simulink model "finalmodel1"  (R2024b)
(part 7 of 9)

Yingli Energy (China) YL345D-36b | Yingli Energy (China) YL350D-36b | Yingli Energy (China) YL355D-36b | Yingli Energy (China) YL360D-36b | YOCASOL PCA200-C04 | YOCASOL PCB200-C21 | YOCASOL PCA205-C04 | YOCASOL PCB205-C21 | YOCASOL PCA210-C04 | YOCASOL PCB210-C21 | Yunnan Tianda Photovoltaic TD160M5 | Yunnan Tianda Photovoltaic TD165M5 | Yunnan Tianda Photovoltaic TD170M5 | Yunnan Tianda Photovoltaic TD175M5 | Yunnan Tianda Photovoltaic TD180M5 | Zebra Energy ZBR-185M5 | Zebra Energy ZBR-190M5 | Zebra Energy ZBR-195M5 | Zebra Energy ZBR-200M5 | Zebra Energy ZBR-200P | Zebra Energy ZBR-210P | Zebra Energy ZBR-220P | Zebra Energy ZBR-230P | Zebra Energy ZBR-235P | Zebra Energy ZBR-240MA | Zebra Energy ZBR-240PA | Zebra Energy ZBR-245MA | Zebra Energy ZBR-250MA | Zebra Energy ZBR-250P | Zebra Energy ZBR-255M | Zebra Energy ZBR-260P | Zebra Energy ZBR-270P | Zebra Energy ZBR-280P | Zebra Energy ZBR-285P | Zebra Energy ZBR-290M | Zebra Energy ZBR-290P | Zebra Energy ZBR-295M | Zebra Energy ZBR-295P | Zebra Energy ZBR-300M | Zebra Energy ZBR-300P | Zebra Energy ZBR-305M | Zebra Energy ZBR-310M | Zerquest Solar Zp170 | Zhangjiagang City SEG PV SEGM5-72 170W | Zhangjiagang City SEG PV SEGM5-72 175W | Zhangjiagang City SEG PV SEGM5-72 180W | Zhangjiagang City SEG PV SEGM5-72 185W | Zhangjiagang City SEG PV SEGM5-72 190W | Zhangjiagang City SEG PV SEGM6-54 190W | Zhangjiagang City SEG PV SEGM5-72 195W | Zhangjiagang City SEG PV SEGM6-54 195W | Zhangjiagang City SEG PV SEGM6-54 200W | Zhangjiagang City SEG PV SEGM6-60 200W | Zhangjiagang City SEG PV SEGM6-54 205W | Zhangjiagang City SEG PV SEGM6-60 205W | Zhangjiagang City SEG PV SEGM6-54 210W | Zhangjiagang City SEG PV SEGM6-60 210W | Zhangjiagang City SEG PV SEGM6-60 215W | Zhangjiagang City SEG PV SEGM6-60 220W | Zhangjiagang City SEG PV SEGM6-60 225W | Zhangjiagang City SEG PV SEGM5-96 230W | Zhangjiagang City SEG PV SEGM6-60 230W | Zhangjiagang City SEG PV SEGM5-96 235W | Zhangjiagang City SEG PV SEGM6-60 235W | Zhangjiagang City SEG PV SEGM5-96 240W | Zhangjiagang City SEG PV SEGM6-60 240W | Zhangjiagang City SEG PV SEGM5-96 245W | Zhangjiagang City SEG PV SEGM5-96 250W | Zhangjiagang City SEG PV SEGM5-96 255W | Zhangjiagang City SEG PV SEGM6-72 255W | Zhangjiagang City SEG PV SEGP6-72 255W | Zhangjiagang City SEG PV SEGM6-72 260W | Zhangjiagang City SEG PV SEGP6-72 260W | Zhangjiagang City SEG PV SEGM6-72 265W | Zhangjiagang City SEG PV SEGP6-72 265W | Zhangjiagang City SEG PV SEGM6-72 270W | Zhangjiagang City SEG PV SEGP6-72 270W | Zhangjiagang City SEG PV SEGM6-72 275W | Zhangjiagang City SEG PV SEGP6-72 275W | Zhangjiagang City SEG PV SEGM6-72 280W | Zhangjiagang City SEG PV SEGP6-72 280W | Zhangjiagang City SEG PV SEGM6-72 285W | Zhangjiagang City SEG PV SEGP6-72 285W | Zhangjiagang City SEG PV SEGM6-72 290W | Zhangjiagang City SEG PV SEGP6-72 290W | Zhangjiagang City SEG PV SEGM6-72 295W | Zhangjiagang City SEG PV SEGP6-72 295W | Zhangjiagang City SEG PV SEGM6-72 300W | Zhangjiagang City SEG PV SEGP6-72 300W | Zhangjiagang City Sunlink PV SEGP6-54-195 | Zhangjiagang City Sunlink PV SEGP6-54-200 | Zhangjiagang City Sunlink PV SEGP6-54-205 | Zhangjiagang City Sunlink PV SEGP6-60-220 | Zhangjiagang City Sunlink PV SEGP6-60-225 | Zhangjiagang City Sunlink PV SEGP6-60-230 | Zhejiang ERA Solar Technology ESPSA-170 | Zhejiang ERA Solar Technology ESPSA-175 | Zhejiang ERA Solar Technology ESPSA-180 | Zhejiang Global Photovoltaic Technology GSM-155 | Zhejiang Global Photovoltaic Technology GSM-160 | Zhejiang Global Photovoltaic Technology GSM-165 | Zhejiang Global Photovoltaic Technology GSM-170 | Zhejiang Global Photovoltaic Technology GSM-175 | Zhejiang Global Photovoltaic Technology GSM-180 | Zhejiang Global Photovoltaic Technology GSP-230 | Zhejiang Global Photovoltaic Technology GSM-235 | Zhejiang Global Photovoltaic Technology GSP-235 | Zhejiang Global Photovoltaic Technology GSM-240 | Zhejiang Global Photovoltaic Technology GSP-240 | Zhejiang Global Photovoltaic Technology GSM-245 | Zhejiang Global Photovoltaic Technology GSM-250 | Zhejiang Global Photovoltaic Technology GSP-265 | Zhejiang Global Photovoltaic Technology GSP-270 | Zhejiang Global Photovoltaic Technology GSM-275 | Zhejiang Global Photovoltaic Technology GSP-275 | Zhejiang Global Photovoltaic Technology GSM-280 | Zhejiang Global Photovoltaic Technology GSP-280 | Zhejiang Global Photovoltaic Technology GSM-285 | Zhejiang Global Photovoltaic Technology GSP-285 | Zhejiang Global Photovoltaic Technology GSM-290 | Zhejiang Global Photovoltaic Technology GSM-295 | Zhejiang Global Photovoltaic Technology GSM-300 | Zhejiang Global Photovoltaic Technology GSM-305 | Zhejiang Guangyi Optical Energy Technology GYP-150M | Zhejiang Guangyi Optical Energy Technology GYP-170P | Zhejiang Guangyi Optical Energy Technology GYP-175P | Zhejiang Guangyi Optical Energy Technology GYP-180M | Zhejiang Guangyi Optical Energy Technology GYP-180P | Zhejiang Guangyi Optical Energy Technology GYP-185M | Zhejiang Guangyi Optical Energy Technology GYP-185P | Zhejiang Guangyi Optical Energy Technology GYP-190P | Zhejiang Guangyi Optical Energy Technology GYP-200P | Zhejiang Guangyi Optical Energy Technology GYP-210P | Zhejiang Guangyi Optical Energy Technology GYP-220P | Zhejiang Guangyi Optical Energy Technology GYP-225P | Zhejiang Guangyi Optical Energy Technology GYP-230M | Zhejiang Guangyi Optical Energy Technology GYP-230P | Zhejiang Guangyi Optical Energy Technology GYP-235M | Zhejiang Guangyi Optical Energy Technology GYP-240M | Zhejiang Guangyi Optical Energy Technology GYP-245M | Zhejiang Guangyi Optical Energy Technology GYP-250M | Zhejiang Guangyi Optical Energy Technology GYP-265P | Zhejiang Guangyi Optical Energy Technology GYP-270M | Zhejiang Guangyi Optical Energy Technology GYP-270P | Zhejiang Guangyi Optical Energy Technology GYP-280M | Zhejiang Guangyi Optical Energy Technology GYP-280P | Zhejiang Guangyi Optical Energy Technology GYP-285P | Zhejiang Guangyi Optical Energy Technology GYP-290M | Zhejiang Jingshang New Energy Technology STS-6M-145P-36 | Zhejiang Jingshang New Energy Technology STS-6M-150P-36 | Zhejiang Jingshang New Energy Technology STS-6M-155P-36 | Zhejiang Jingshang New Energy Technology STS-6M-185P-48 | Zhejiang Jingshang New Energy Technology STS-6M-190P-48 | Zhejiang Jingshang New Energy Technology STS-6M-195P-48 | Zhejiang Jingshang New Energy Technology STS-6M-200P-48 | Zhejiang Jingshang New Energy Technology STS-6M-210P-54 | Zhejiang Jingshang New Energy Technology STS-6M-215P-54 | Zhejiang Jingshang New Energy Technology STS-6M-220P-54 | Zhejiang Jingshang New Energy Technology STS-6M-225P-54 | Zhejiang Jingshang New Energy Technology STS-6M-230P-54 | Zhejiang Jingshang New Energy Technology STS-6M-235P-60 | Zhejiang Jingshang New Energy Technology STS-6M-240P-60 | Zhejiang Jingshang New Energy Technology STS-6M-245P-60 | Zhejiang Jingshang New Energy Technology STS-6M-250P-60 | Zhejiang Jingshang New Energy Technology STS-6M-255P-60 | Zhejiang Jingshang New Energy Technology STS-6M-260P-60 | Zhejiang Jingshang New Energy Technology STS-6M-265P-60 | Zhejiang Jingshang New Energy Technology STS-6M-270P-72 | Zhejiang Jingshang New Energy Technology STS-6M-275P-72 | Zhejiang Jingshang New Energy Technology STS-6M-280P-72 | Zhejiang Jingshang New Energy Technology STS-6M-285P-72 | Zhejiang Jingshang New Energy Technology STS-6M-290P-72 | Zhejiang Jingshang New Energy Technology STS-6M-295P-72 | Zhejiang Jingshang New Energy Technology STS-6M-300P-72 | Zhejiang Jingshang New Energy Technology STS-6M-305P-72 | Zhejiang Jingshang New Energy Technology STS-6M-310P-72 | Zhejiang Jingshang New Energy Technology STS-6M-315P-72 | Zhejiang Jingshang New Energy Technology STS-6M-320P-72 | Zhejiang Jiutai New Energy JTM175-72M | Zhejiang Jiutai New Energy JTM180-72M | Zhejiang Jiutai New Energy JTM185-72M | Zhejiang Jiutai New Energy JTM200-60P | Zhejiang Jiutai New Energy JTM205-60P | Zhejiang Jiutai New Energy JTM210-60P | Zhejiang Jiutai New Energy JTM215-60P | Zhejiang Jiutai New Energy JTM220-60P | Zhejiang Jiutai New Energy JTM225-60P | Zhejiang Jiutai New Energy JTM230-60P | Zhejiang Jiutai New Energy JTM235-60P | Zhejiang Jiutai New Energy JTM240-60P | Zhejiang Jiutai New Energy JTM270-72P | Zhejiang Jiutai New Energy JTM275-72P | Zhejiang Jiutai New Energy JTM280-72P | Zhejiang Jiutai New Energy JTM285-72P | Zhejiang Kingdom Solar Energy Technic KD-M160 | Zhejiang Kingdom Solar Energy Technic KD-M165 | Zhejiang Kingdom Solar Energy Technic KD-M170 | Zhejiang Kingdom Solar Energy Technic KD-M175 | Zhejiang Kingdom Solar Energy Technic KD-M180 | Zhejiang Kingdom Solar Energy Technic KD-M185 | Zhejiang Kingdom Solar Energy Technic KD-M190 | Zhejiang Kingdom Solar Energy Technic KD-M195 | Zhejiang Kingdom Solar Energy Technic KD-M200 | Zhejiang Kingdom Solar Energy Technic KD-P200 | Zhejiang Kingdom Solar Energy Technic KD-P205 | Zhejiang Kingdom Solar Energy Technic KD-P210 | Zhejiang Kingdom Solar Energy Technic KD-P215 | Zhejiang Kingdom Solar Energy Technic KD-P220 | Zhejiang Kingdom Solar Energy Technic KD-P225 | Zhejiang Kingdom Solar Energy Technic KD-P230 | Zhejiang Kingdom Solar Energy Technic KD-P235 | Zhejiang Kingdom Solar Energy Technic KD-P240 | Zhejiang Kingdom Solar Energy Technic KD-P245 | Zhejiang Kingdom Solar Energy Technic KD-P250 | Zhejiang Kingdom Solar Energy Technic KD-P255 | Zhejiang Kingdom Solar Energy Technic KD-P260 | Zhejiang Kingdom Solar Energy Technic KD-P265 | Zhejiang Kingdom Solar Energy Technic KD-P270 | Zhejiang Kingdom Solar Energy Technic KD-P275 | Zhejiang Kingdom Solar Energy Technic KD-P280 | Zhejiang Kingdom Solar Energy Technic KD-P285 | Zhejiang Kingdom Solar Energy Technic KD-P290 | Zhejiang Kingdom Solar Energy Technic KD-P295 | Zhejiang Kingdom Solar Energy Technic KD-P300 | Zhejiang Shinew Photoelectronic Technology XH-72M-185 | Zhejiang Shinew Photoelectronic Technology XH-72M-190 | Zhejiang Shinew Photoelectronic Technology XH-60P-230 | Zhejiang Shinew Photoelectronic Technology XH-60P-235 | Zhejiang Shinew Photoelectronic Technology XH-72P-280 | ZheJiang SOCO Technology SC180M-24/P | ZheJiang SOCO Technology SC230M-24/J | ZheJiang SOCO Technology SC230P-24/B | ZheJiang SOCO Technology SC275P-24/A | ZheJiang SOCO Technology SC280M-24/H | Zhejiang Sunflower Light Energy Science & Technology SF125x125-72-M-150W | Zhejiang Sunflower Light Energy Science & Technology SF125x125-72-M-155W | Zhejiang Sunflower Light Energy Science & Technology SF125x125-72-M-160W | Zhejiang Sunflower Light Energy Science & Technology SF125x125-72-M-165W | Zhejiang Sunflower Light Energy Science & Technology SF125x125-72-M-170W | Zhejiang Sunflower Light Energy Science & Technology SF125x125-72-M-175W | Zhejiang Sunflower Light Energy Science & Technology SF125x125-72-M-180W | Zhejiang Sunflower Light Energy Science & Technology SF125x125-72-M-185W | Zhejiang Sunflower Light Energy Science & Technology SF156x156-60-M-200W | Zhejiang Sunflower Light Energy Science & Technology SF156x156-60-P-200W | Zhejiang Sunflower Light Energy Science & Technology SF156x156-60-M-205W | Zhejiang Sunflower Light Energy Science & Technology SF156x156-60-P-205W | Zhejiang Sunflower Light Energy Science & Technology SF156x156-60-M-210W | Zhejiang Sunflower Light Energy Science & Technology SF156x156-60-P-210W | Zhejiang Sunflower Light Energy Science & Technology SF156x156-60-M-215W | Zhejiang Sunflower Light Energy Science & Technology SF156x156-60-P-215W | Zhejiang Sunflower Light Energy Science & Technology SF156x156-60-M-220W | Zhejiang Sunflower Light Energy Science & Technology SF156x156-60-P-220W | Zhejiang Sunflower Light Energy Science & Technology SF156x156-60-M-225W | Zhejiang Sunflower Light Energy Science & Technology SF156x156-60-P-225W | Zhejiang Sunflower Light Energy Science & Technology SF156x156-60-M-230W | Zhejiang Sunflower Light Energy Science & Technology SF156x156-60-P-230W | Zhejiang Sunflower Light Energy Science & Technology SF156x156-60-M-235W | Zhejiang Sunflower Light Energy Science & Technology SF156x156-60-M-240W | Zhejiang Trunsun Solar Co._ Ltd. TSP255-60 | Zhejiang Trunsun Solar Co._ Ltd. TSM260-60 | Zhejiang Trunsun Solar Co._ Ltd. TSP260-60 | Zhejiang Trunsun Solar Co._ Ltd. TSM265-60 | Zhejiang Trunsun Solar Co._ Ltd. TSP265-60 | Zhejiang Trunsun Solar Co._ Ltd. TSM270-60 | Zhejiang Trunsun Solar Co._ Ltd. TSP270-60 | Zhejiang Trunsun Solar Co._ Ltd. TSM275-60 | Zhejiang Trunsun Solar Co._ Ltd. TSP275-60 | Zhejiang Trunsun Solar Co._ Ltd. TSP305-72 | Zhejiang Trunsun Solar Co._ Ltd. TSM310-72 | Zhejiang Trunsun Solar Co._ Ltd. TSP310-72 | Zhejiang Trunsun Solar Co._ Ltd. TSM315-72 | Zhejiang Trunsun Solar Co._ Ltd. TSP315-72 | Zhejiang Trunsun Solar Co._ Ltd. TSM320-72 | Zhejiang Trunsun Solar Co._ Ltd. TSP320-72 | Zhejiang Trunsun Solar Co._ Ltd. TSM325-72 | Zhejiang Trunsun Solar Co._ Ltd. TSP325-72 | Zhejiang Trunsun Solar Co._ Ltd. TSM330-72 | Zhejiang Trunsun Solar Co._ Ltd. TSP330-72 | Zhejiang Trunsun Solar Co._ Ltd. TSP335-72 | Zhejiang Wanxiang Solar WXS175P | Zhejiang Wanxiang Solar WXS175S | Zhejiang Wanxiang Solar WXS180P | Zhejiang Wanxiang Solar WXS180S | Zhejiang Wanxiang Solar WXS185P | Zhejiang Wanxiang Solar WXS185S | Zhejiang Wanxiang Solar WXS190P | Zhejiang Wanxiang Solar WXS200P | Zhejiang Wanxiang Solar WXS205P | Zhejiang Wanxiang Solar WXS210P | Zhejiang Wanxiang Solar WXS215P | Zhejiang Wanxiang Solar WXS220P | Zhejiang Wanxiang Solar WXS225P | Zhejiang Wanxiang Solar WXS230P | Zhejiang Wanxiang Solar WXS235P | Zhejiang Wanxiang Solar WXS240P | Zhejiang Wanxiang Solar WXS245P | Zhejiang Wanxiang Solar WXS250P | Zhejiang Wanxiang Solar WXS255P | Zhejiang Wanxiang Solar WXS260P | Zhejiang Wanxiang Solar WXS265P | Zhejiang Wanxiang Solar WXS270P | Zhejiang Wanxiang Solar WXS275P | Zhejiang Wanxiang Solar WXS280P | Znshine PV-Tech ZXM5-72-175/MS | Znshine PV-Tech ZXM5-72-180/MS | Znshine PV-Tech ZXM5-72-185/MS | Znshine PV-Tech ZXM5-72-190/MS | Znshine PV-Tech ZXM5-72-195/MS | Znshine PV-Tech ZXM5-72-200/MS | Znshine PV-Tech ZXP6-60-220/P | Znshine PV-Tech ZXP6-60-225/P | Znshine PV-Tech ZXP6-60-230/P | Znshine PV-Tech ZXP6-60-235/P | Znshine PV-Tech ZXP6-D60-235/P | Znshine PV-Tech ZXM6-D60-240/M | Znshine PV-Tech ZXP6-60-240/P | Znshine PV-Tech ZXP6-D60-240/P | Znshine PV-Tech ZXM5-96-245/MS | Znshine PV-Tech ZXM6-D60-245/M | Znshine PV-Tech ZXP6-60-245/P | Znshine PV-Tech ZXP6-D60-245/P | Znshine PV-Tech ZXM5-96-250/MS | Znshine PV-Tech ZXM6-D60-250/M | Znshine PV-Tech ZXP6-D60-250/P | Znshine PV-Tech ZXM5-96-255/MS | Znshine PV-Tech ZXM6-D60-255/M | Znshine PV-Tech ZXP6-D60-255/P | Znshine PV-Tech ZXM5-96-260/MS | Znshine PV-Tech ZXM6-D60-260/M | Znshine PV-Tech ZXM5-96-265/MS | Znshine PV-Tech ZXP6-72-265/P | Znshine PV-Tech ZXM5-96-270/MS | Znshine PV-Tech ZXP6-72-270/P | Znshine PV-Tech ZXM5-96-275/MS | Znshine PV-Tech ZXP6-72-275/P | Znshine PV-Tech ZXP6-72-280/P | Znshine PV-Tech ZXP6-72-285/P | Znshine PV-Tech ZXP6-72-290/P | Znshine PV-Tech ZXP6-72-295/P | Zytech Engineering Technology ZT170S | Zytech Engineering Technology ZT175S | Zytech Engineering Technology ZT180S | Zytech Engineering Technology ZT185S | Zytech Engineering Technology ZT190S | Zytech Solar ZT145P | Zytech Solar ZT150P | Zytech Solar ZT155P | Zytech Solar ZT185P | Zytech Solar ZT190P | Zytech Solar ZT195P | Zytech Solar ZT200P | Zytech Solar ZT210P | Zytech Solar ZT215P | Zytech Solar ZT220P | Zytech Solar ZT225P | Zytech Solar ZT230P | Zytech Solar ZT235P | Zytech Solar ZT240P | Zytech Solar ZT245P | Zytech Solar ZT250P | Zytech Solar ZT255P | Zytech Solar ZT260P | Zytech Solar ZT265P | Zytech Solar ZT270P | Zytech Solar ZT275P | Zytech Solar ZT280P | Zytech Solar ZT285P | Zytech Solar ZT290P | Zytech Solar ZT295P | Zytech Solar ZT300P | Zytech Solar ZT305P | Zytech Solar ZT310P | Zytech Solar ZT315P | Zytech Solar ZT320P
      mask Callback ModuleName: PVArrayCback(gcb)
      mask Callback RobustModel: PVArrayCback(gcb)
      mask Callback BAL: PVArrayCback(gcb)
      mask DialogControl ParameterTabVar0 Prompt: Parameters
      mask DialogControl ArrayData Prompt: Array data
      mask DialogControl Display Prompt: Display  I-V and P-V characteristics of ...
      mask DialogControl PlotButton Prompt: Plot
      mask DialogControl PlotButton Callback: PVArrayPlot(gcb,'detailed')
      mask DialogControl ManufacturerData Prompt: Module data
      mask DialogControl ModelParameters Prompt: Model parameters
      mask DialogControl Advanced Prompt: Advanced
      mask Display:
      | port_label('input',1,'Ir')
      | switch WantBlockChoice{1}
      |     case 'Discrete DSS Diode Rsh'
      |     otherwise
      |         port_label('input',2,'T')
      | end
      | 
      | port_label('output',1,'m')
      | port_label('output',1,'m')
      | port_label('Rconn',1,'+')
      | port_label('Rconn',2,'-')
  PWM Generator (2-Level) : spsPWMGenerator2LevelLib/PWM Generator (2-Level)  ModulatorType=Three-phase bridge (6 pulses)  ModulatorMode=Synchronized  Fc=27*60  Pc=90  nF=27  MinMax="[ -1  1 ]"  SamplingTechnique=Natural  ModulatingSignals=off  m=0.8  Freq=60  Phase=0  Ts=SampleTime  ShowCarrierOutport=off
      link override Modulator type/One Three Phase Bridge/P: SampleTime=SampleTime
      link override P: SampleTime=SampleTime
      link override Reference signal/External/Uref: SampleTime=SampleTime
      link override Uref: SampleTime=SampleTime
      link override wt: SampleTime=SampleTime
  "PWM Generator (DC - DC) " : spsPWMGeneratorDCDCLib/PWM Generator (DC-DC)  Fsw=5e3  Ts=SampleTime
      link override D: SampleTime=SampleTime
      link override Sawtooth Generator: Ts=SampleTime
      link override Sawtooth Generator/Model/Constant2: SampleTime=SampleTime
      link override Sawtooth Generator/Model/Constant3: SampleTime=SampleTime
      link override Sawtooth Generator/Model/Digital Clock: SampleTime=SampleTime
  "Power (3ph, Instantaneous)" : spsPower3phInstantaneousLib/Power (3ph, Instantaneous)
  Product : Product  SampleTime=SampleTime
  Repeating Sequence1 : simulink/Sources/Repeating Sequence  rep_seq_t=[0 0.00005 0.0001]  rep_seq_y=[-1 1 -1]
  Scope : Scope
  Scope1 : Scope  NumInputPorts=2
  Scope2 : Scope  NumInputPorts=2
  Scope4 : Scope
  Scope5 : Scope  NumInputPorts=2
  Signal Builder2 : Subsystem  Tag=STV Subsys  Commented=on  LoadFcn=sigbuilder_block('load');  StartFcn=sigbuilder_block('start');  StopFcn=sigbuilder_block('stop');  ClipboardFcn=sigbuilder_block('clipboard');  mask(Sigbuilder block){tuvar=[0:10]}
      mask help: Simulink:masks:SigbuilderBlock_MD
      mask init:
      | if ~strcmp(get_param(bdroot(gcbh),'SimulationStatus'),'stopped') tuvar = sigbuilder_block('maskInit'); end
      settings: CopyFcn=sigbuilder_block('copy');  DeleteFcn=sigbuilder_block('delete');  ModelCloseFcn=sigbuilder_block('modelClose');  PreSaveFcn=sigbuilder_block('preSave');  PauseFcn=sigbuilder_block('pause');  ContinueFcn=sigbuilder_block('continue');  NameChangeFcn=sigbuilder_block('namechange');  OpenFcn=sigbuilder_block('open',[220.2 153.6 550.8 361.2 ]);  CloseFcn=sigbuilder_block('close');
      mask Display: plot(0, 0, 100, 100,[2, 2, 32, 32, 2], [68, 8, 8, 68, 68],[32, 2], [38, 38], [32, 19, 2],[53, 60, 44], [32, 17, 17, 2],[16, 16, 31, 31]);txt = getActiveGroup(gcbh);text(2, 100, txt,'verticalAlignment', 'top');
  Stop simulation if loss of synchronism : Stop  Commented=on
  Sum{1..3,7} (4 alike) : Sum  Inputs=|+-  SampleTime=SampleTime
  Sum{4..6,8} (4 alike) : Sum  Inputs=|++  SampleTime=SampleTime
  THD : spsTHDLib/THD  Freq=50  Ts=SampleTime
      link override In: SampleTime=SampleTime
      link override Mean: Ts=SampleTime
      link override Mean/In: SampleTime=SampleTime
      link override Mean/Mean: SampleTime=SampleTime
      link override Mean/Model/Digital  Clock: SampleTime=SampleTime
      link override Mean/Model/Discrete Variable Time Delay: Ts=SampleTime
      link override Mean/Model/Discrete Variable Time Delay/D: SampleTime=SampleTime
      link override Mean/Model/Discrete Variable Time Delay/In: SampleTime=SampleTime
      link override Mean/Model/Discrete Variable Time Delay/Out: SampleTime=SampleTime
      link override Mean/Model/Integ4: SampleTime=SampleTime
      link override Mean/Model/K1: SampleTime=SampleTime
      link override Mean/Model/K2: SampleTime=SampleTime
      link override Mean/Model/Relational Operator: SampleTime=SampleTime
      link override Mean/Model/Unit Delay: SampleTime=SampleTime
      link override Mean/Model/Unit Delay1: SampleTime=SampleTime
      link override RMS1: Ts=SampleTime
      link override RMS1/In: SampleTime=SampleTime
      link override RMS1/RMS: SampleTime=SampleTime
      link override RMS1/RMS /Fourier1: Ts=SampleTime
      link override RMS1/RMS /Fourier1/In: SampleTime=SampleTime
      link override RMS1/RMS /Fourier1/Mag: SampleTime=SampleTime
      link override RMS1/RMS /Fourier1/Mean: Ts=SampleTime
      link override RMS1/RMS /Fourier1/Mean value1: Ts=SampleTime
      link override RMS1/RMS /Fourier1/Mean value1/In: SampleTime=SampleTime
      link override RMS1/RMS /Fourier1/Mean value1/Mean: SampleTime=SampleTime
      link override RMS1/RMS /Fourier1/Mean value1/Model/Digital  Clock: SampleTime=SampleTime
      link override RMS1/RMS /Fourier1/Mean value1/Model/Discrete Variable Time Delay: Ts=SampleTime
      link override RMS1/RMS /Fourier1/Mean value1/Model/Discrete Variable Time Delay/D: SampleTime=SampleTime
      link override RMS1/RMS /Fourier1/Mean value1/Model/Discrete Variable Time Delay/In: SampleTime=SampleTime
      link override RMS1/RMS /Fourier1/Mean value1/Model/Discrete Variable Time Delay/Out: SampleTime=SampleTime
      link override RMS1/RMS /Fourier1/Mean value1/Model/Integ4: SampleTime=SampleTime
      link override RMS1/RMS /Fourier1/Mean value1/Model/K1: SampleTime=SampleTime
      link override RMS1/RMS /Fourier1/Mean value1/Model/K2: SampleTime=SampleTime
      link override RMS1/RMS /Fourier1/Mean value1/Model/Relational Operator: SampleTime=SampleTime
      link override RMS1/RMS /Fourier1/Mean value1/Model/Unit Delay: SampleTime=SampleTime
      link override RMS1/RMS /Fourier1/Mean value1/Model/Unit Delay1: SampleTime=SampleTime
      link override RMS1/RMS /Fourier1/Mean/In: SampleTime=SampleTime
      link override RMS1/RMS /Fourier1/Mean/Mean: SampleTime=SampleTime
      link override RMS1/RMS /Fourier1/Mean/Model/Digital  Clock: SampleTime=SampleTime
      link override RMS1/RMS /Fourier1/Mean/Model/Discrete Variable Time Delay: Ts=SampleTime
      link override RMS1/RMS /Fourier1/Mean/Model/Discrete Variable Time Delay/D: SampleTime=SampleTime
      link override RMS1/RMS /Fourier1/Mean/Model/Discrete Variable Time Delay/In: SampleTime=SampleTime
      link override RMS1/RMS /Fourier1/Mean/Model/Discrete Variable Time Delay/Out: SampleTime=SampleTime
      link override RMS1/RMS /Fourier1/Mean/Model/Integ4: SampleTime=SampleTime
      link override RMS1/RMS /Fourier1/Mean/Model/K1: SampleTime=SampleTime
      link override RMS1/RMS /Fourier1/Mean/Model/K2: SampleTime=SampleTime
      link override RMS1/RMS /Fourier1/Mean/Model/Relational Operator: SampleTime=SampleTime
      link override RMS1/RMS /Fourier1/Mean/Model/Unit Delay: SampleTime=SampleTime
      link override RMS1/RMS /Fourier1/Mean/Model/Unit Delay1: SampleTime=SampleTime
      link override RMS1/RMS /Fourier1/Phase: SampleTime=SampleTime
      link override RMS1/RMS /Fourier1/cos(wt): SampleTime=SampleTime
      link override RMS1/RMS /Fourier1/sin(wt): SampleTime=SampleTime
      link override RMS1/TrueRMS /Mean value: Ts=SampleTime
      link override RMS1/TrueRMS /Mean value/In: SampleTime=SampleTime
      link override RMS1/TrueRMS /Mean value/Mean: SampleTime=SampleTime
      link override RMS1/TrueRMS /Mean value/Model/Digital  Clock: SampleTime=SampleTime
      link override RMS1/TrueRMS /Mean value/Model/Discrete Variable Time Delay: Ts=SampleTime
      link override RMS1/TrueRMS /Mean value/Model/Discrete Variable Time Delay/D: SampleTime=SampleTime
      link override RMS1/TrueRMS /Mean value/Model/Discrete Variable Time Delay/In: SampleTime=SampleTime
      link override RMS1/TrueRMS /Mean value/Model/Discrete Variable Time Delay/Out: SampleTime=SampleTime
      link override RMS1/TrueRMS /Mean value/Model/Integ4: SampleTime=SampleTime
      link override RMS1/TrueRMS /Mean value/Model/K1: SampleTime=SampleTime
      link override RMS1/TrueRMS /Mean value/Model/K2: SampleTime=SampleTime
      link override RMS1/TrueRMS /Mean value/Model/Relational Operator: SampleTime=SampleTime
      link override RMS1/TrueRMS /Mean value/Model/Unit Delay: SampleTime=SampleTime
      link override RMS1/TrueRMS /Mean value/Model/Unit Delay1: SampleTime=SampleTime
      link override RMS2: Ts=SampleTime
      link override RMS2/In: SampleTime=SampleTime
      link override RMS2/RMS: SampleTime=SampleTime
      link override RMS2/RMS /Fourier1: Ts=SampleTime
      link override RMS2/RMS /Fourier1/In: SampleTime=SampleTime
      link override RMS2/RMS /Fourier1/Mag: SampleTime=SampleTime
      link override RMS2/RMS /Fourier1/Mean: Ts=SampleTime
      link override RMS2/RMS /Fourier1/Mean value1: Ts=SampleTime
      link override RMS2/RMS /Fourier1/Mean value1/In: SampleTime=SampleTime
      link override RMS2/RMS /Fourier1/Mean value1/Mean: SampleTime=SampleTime
      link override RMS2/RMS /Fourier1/Mean value1/Model/Digital  Clock: SampleTime=SampleTime
      link override RMS2/RMS /Fourier1/Mean value1/Model/Discrete Variable Time Delay: Ts=SampleTime
      link override RMS2/RMS /Fourier1/Mean value1/Model/Discrete Variable Time Delay/D: SampleTime=SampleTime
      link override RMS2/RMS /Fourier1/Mean value1/Model/Discrete Variable Time Delay/In: SampleTime=SampleTime
      link override RMS2/RMS /Fourier1/Mean value1/Model/Discrete Variable Time Delay/Out: SampleTime=SampleTime
      link override RMS2/RMS /Fourier1/Mean value1/Model/Integ4: SampleTime=SampleTime
      link override RMS2/RMS /Fourier1/Mean value1/Model/K1: SampleTime=SampleTime
      link override RMS2/RMS /Fourier1/Mean value1/Model/K2: SampleTime=SampleTime
      link override RMS2/RMS /Fourier1/Mean value1/Model/Relational Operator: SampleTime=SampleTime
      link override RMS2/RMS /Fourier1/Mean value1/Model/Unit Delay: SampleTime=SampleTime
      link override RMS2/RMS /Fourier1/Mean value1/Model/Unit Delay1: SampleTime=SampleTime
      link override RMS2/RMS /Fourier1/Mean/In: SampleTime=SampleTime
      link override RMS2/RMS /Fourier1/Mean/Mean: SampleTime=SampleTime
      link override RMS2/RMS /Fourier1/Mean/Model/Digital  Clock: SampleTime=SampleTime
      link override RMS2/RMS /Fourier1/Mean/Model/Discrete Variable Time Delay: Ts=SampleTime
      link override RMS2/RMS /Fourier1/Mean/Model/Discrete Variable Time Delay/D: SampleTime=SampleTime
      link override RMS2/RMS /Fourier1/Mean/Model/Discrete Variable Time Delay/In: SampleTime=SampleTime
      link override RMS2/RMS /Fourier1/Mean/Model/Discrete Variable Time Delay/Out: SampleTime=SampleTime
      link override RMS2/RMS /Fourier1/Mean/Model/Integ4: SampleTime=SampleTime
      link override RMS2/RMS /Fourier1/Mean/Model/K1: SampleTime=SampleTime
      link override RMS2/RMS /Fourier1/Mean/Model/K2: SampleTime=SampleTime
      link override RMS2/RMS /Fourier1/Mean/Model/Relational Operator: SampleTime=SampleTime
      link override RMS2/RMS /Fourier1/Mean/Model/Unit Delay: SampleTime=SampleTime
      link override RMS2/RMS /Fourier1/Mean/Model/Unit Delay1: SampleTime=SampleTime
      link override RMS2/RMS /Fourier1/Phase: SampleTime=SampleTime
      link override RMS2/RMS /Fourier1/cos(wt): SampleTime=SampleTime
      link override RMS2/RMS /Fourier1/sin(wt): SampleTime=SampleTime
      link override RMS2/TrueRMS /Mean value: Ts=SampleTime
      link override RMS2/TrueRMS /Mean value/In: SampleTime=SampleTime
      link override RMS2/TrueRMS /Mean value/Mean: SampleTime=SampleTime
      link override RMS2/TrueRMS /Mean value/Model/Digital  Clock: SampleTime=SampleTime
      link override RMS2/TrueRMS /Mean value/Model/Discrete Variable Time Delay: Ts=SampleTime
      link override RMS2/TrueRMS /Mean value/Model/Discrete Variable Time Delay/D: SampleTime=SampleTime
      link override RMS2/TrueRMS /Mean value/Model/Discrete Variable Time Delay/In: SampleTime=SampleTime
      link override RMS2/TrueRMS /Mean value/Model/Discrete Variable Time Delay/Out: SampleTime=SampleTime
      link override RMS2/TrueRMS /Mean value/Model/Integ4: SampleTime=SampleTime
      link override RMS2/TrueRMS /Mean value/Model/K1: SampleTime=SampleTime
      link override RMS2/TrueRMS /Mean value/Model/K2: SampleTime=SampleTime
      link override RMS2/TrueRMS /Mean value/Model/Relational Operator: SampleTime=SampleTime
      link override RMS2/TrueRMS /Mean value/Model/Unit Delay: SampleTime=SampleTime
      link override RMS2/TrueRMS /Mean value/Model/Unit Delay1: SampleTime=SampleTime
      link override THD: SampleTime=SampleTime
  Three-Phase Parallel RLC Load : spsThreePhaseParallelRLCLoadLib/Three-Phase Parallel RLC Load  LConnTagsString=A|B|C  Configuration=Y (grounded)  NominalVoltage=230e3  Vabc=[1e3 1e3 1e3]  Vabcp=[1e3 1e3 1e3]  NominalFrequency=60  UnbalancedPower=off  ActivePower=30e6  InductivePower=0  CapacitivePower=0  Pabc=[10e3 9e3 11e3]  QLabc=[100 90 110]  QCabc=[100 90 110]  Pabcp=[10e3 9e3 11e3]  QLabcp=[100 90 110]  QCabcp=[100 90 110]  Measurements=None  LoadType=constant Z
  Three-Phase Series RLC Branch1 : spsThreePhaseSeriesRLCBranchLib/Three-Phase Series RLC Branch  LConnTagsString=A|B|C  RConnTagsString=A|B|C  BranchType=RL  Resistance=1e-3  Inductance=500e-6  Capacitance=1e-6  Measurements=None
  Three-Phase Series RLC Branch2 : spsThreePhaseSeriesRLCBranchLib/Three-Phase Series RLC Branch  LConnTagsString=A|B|C  RConnTagsString=A|B|C  BranchType=RL  Resistance=1e-3  Inductance=500e-6  Capacitance=1e-6  Measurements=None
  Three-Phase Series RLC Branch3 : spsThreePhaseSeriesRLCBranchLib/Three-Phase Series RLC Branch  LConnTagsString=A|B|C  RConnTagsString=A|B|C  BranchType=RC  Resistance=1  Inductance=500e-6  Capacitance=100e-6  Measurements=None
  Three-Phase Transformer (Two Windings) : spsThreePhaseTransformerTwoWindingsLib/Three-Phase Transformer (Two Windings)  Winding1Connection=Yg  Winding2Connection=Yg  CoreType=Three single-phase transformers  SetSaturation=off  Hysteresis=off  DataFile='hysteresis'  SetInitialFlux=off  Measurements=None  UNITS=pu  NominalPower=[ 200e6 , 60 ]  Winding1=[ 400 , 0.002 , 0.08 ]  Winding2=[ 18e3 , 0.002 , 0.08 ]  Rm=500  Lm=500  L0=0.5  Saturation=[ 0,0 ; 0.0024,1.2 ; 1.0,1.52 ]  InitialFluxes=[ 0.8 , -0.8 , 0.7 ]  BreakLoop=off  DiscreteSolver=Trapezoidal iterative  DataType=off  TransfoNumber=1
  Three-Phase Breaker : spsThreePhaseBreakerLib/Three-Phase Breaker  InitialState=open  SwitchA=on  SwitchB=on  SwitchC=on  SwitchTimes=[50]  External=off  BreakerResistance=0.01  SnubberResistance=1e6  SnubberCapacitance=inf  Measurements=None
      link override Breaker A/Model/C4: SampleTime=SampleTime
      link override Breaker A/Model/Timer: Ts=SampleTime
      link override Breaker A/Model/Timer/Digital Clock: SampleTime=SampleTime
      link override Breaker A/Model/Uswitch: SampleTime=SampleTime
      link override Breaker A/Model/gate: SampleTime=SampleTime
      link override Breaker B/Model/C4: SampleTime=SampleTime
      link override Breaker B/Model/Timer: Ts=SampleTime
      link override Breaker B/Model/Timer/Digital Clock: SampleTime=SampleTime
      link override Breaker B/Model/Uswitch: SampleTime=SampleTime
      link override Breaker B/Model/gate: SampleTime=SampleTime
      link override Breaker C/Model/C4: SampleTime=SampleTime
      link override Breaker C/Model/Timer: Ts=SampleTime
      link override Breaker C/Model/Timer/Digital Clock: SampleTime=SampleTime
      link override Breaker C/Model/Uswitch: SampleTime=SampleTime
      link override Breaker C/Model/gate: SampleTime=SampleTime
      link override Stair Generator: Ts=SampleTime
      link override Stair Generator/Model/Digital Clock: SampleTime=SampleTime
      link override Stair Generator/Model/Look-Up Table: SampleTime=SampleTime
      link override Stair Generator/Out: SampleTime=SampleTime
  Two-Level Converter : spsTwoLevelConverterLib/Two-Level Converter  ModelType=Switching devices  Ron=1e-3  Rs=1e6  Cs=inf  Vforward=[0,0]  Ron_Diode=1e-3  Rs_Diode=1e6  Cs_Diode=inf  Vf_Diode=1e-3  Rs_CurrentSource=inf  Ron_ACsource=1e-3
      settings: LibrarySourceBlock=sps_lib/Power Electronics/Two-Level Converter
  "V_dc " : Scope
  Vabc5_log : ToWorkspace  VariableName=Vabc5_log  SaveFormat=Timeseries  SampleTime=-1
  Vgq : Constant  Value=0  SampleTime=SampleTime
  Voltage Measurement1 : spsVoltageMeasurementLib/Voltage Measurement  PhasorSimulation=off  OutputType=Magnitude  PSBequivalent=0
  Vpcc1_log : ToWorkspace  VariableName=Vpcc1_log  SaveFormat=Timeseries  SampleTime=-1
  abc to Alpha-Beta-Zero : spsabctoAlphaBetaZeroLib/abc to Alpha-Beta-Zero
  abc to Alpha-Beta-Zero1 : spsabctoAlphaBetaZeroLib/abc to Alpha-Beta-Zero
  abc to dq0 : spsabctodq0Lib/abc to dq0  Alignment=90 degrees behind phase A axis
  dq0 to abc : spsdq0toabcLib/dq0 to abc  Alignment=90 degrees behind phase A axis
  load1 : spsThreePhaseParallelRLCLoadLib/Three-Phase Parallel RLC Load  LConnTagsString=A|B|C  Configuration=Y (grounded)  NominalVoltage=(230000)*1.0168  Vabc=[1e3 1e3 1e3]  Vabcp=[1e3 1e3 1e3]  NominalFrequency=60  UnbalancedPower=off  ActivePower=100000000  InductivePower=35000000  CapacitivePower=0  Pabc=[10e3 9e3 11e3]  QLabc=[100 90 110]  QCabc=[100 90 110]  Pabcp=[10e3 9e3 11e3]  QLabcp=[100 90 110]  QCabcp=[100 90 110]  Measurements=None  LoadType=constant PQ
  load2 : spsThreePhaseParallelRLCLoadLib/Three-Phase Parallel RLC Load  LConnTagsString=A|B|C  Configuration=Y (grounded)  NominalVoltage=(230000)*1.00166  Vabc=[1e3 1e3 1e3]  Vabcp=[1e3 1e3 1e3]  NominalFrequency=60  UnbalancedPower=off  ActivePower=125000000  InductivePower=50000000  CapacitivePower=0  Pabc=[10e3 9e3 11e3]  QLabc=[100 90 110]  QCabc=[100 90 110]  Pabcp=[10e3 9e3 11e3]  QLabcp=[100 90 110]  QCabcp=[100 90 110]  Measurements=None  LoadType=constant PQ
  load4 : spsThreePhaseParallelRLCLoadLib/Three-Phase Parallel RLC Load  LConnTagsString=A|B|C  Configuration=Y (grounded)  NominalVoltage=(230000)*1.01715  Vabc=[1e3 1e3 1e3]  Vabcp=[1e3 1e3 1e3]  NominalFrequency=60  UnbalancedPower=off  ActivePower=90000000  InductivePower=30000000  CapacitivePower=0  Pabc=[10e3 9e3 11e3]  QLabc=[100 90 110]  QCabc=[100 90 110]  Pabcp=[10e3 9e3 11e3]  QLabcp=[100 90 110]  QCabcp=[100 90 110]  Measurements=None  LoadType=constant PQ
  powergui : spspowerguiLib/powergui  Priority=1  SimulationMode=Discrete  SampleTime=SampleTime  frequency=60  Iterations=50  frequencyindice=60  Pbase=100e6  ErrMax=1e-4  UnitsV=V  UnitsW=MW  buscounter=0  FunctionMessages=off  echomessages=off  EnableUseOfTLC=off  CurrentSourceSwitches=off  DisableSnubberDevices=off  DisableRonSwitches=off  DisableVfSwitches=off  DisplayEquations=off  AutomaticDiscreteSolvers=off  SolverType=Tustin/Backward Euler (TBE)  Interpol=off  ExternalGateDelay=off  methode=off  Ts=SampleTime  x0status=blocks  SPID=on  SwTol=0  HookPort=off  NonlinearTolerance=1e-4  nMaxIteration=100  ContinueOnMaxIteration=off  RestoreLinks=warning  ResistiveCurrentMeasurement=off  Frange=[0:2:500]  Ylog=off  Xlog=on  ShowGrid=off  save=off  variable=ZData  structure=0  ZoomFFT=off  StartTime=0.0  cycles=1  DisplayStyle=1  fundamental=60  FreqAxis=off  MaxFrequency=1000  frequencyindicesteady=1  RmsSteady=1  display=off
  powergui_auto : spspowerguiLib/powergui  Priority=1  SimulationMode=Discrete  SampleTime=SampleTime  frequency=60  Iterations=50  frequencyindice=60  Pbase=100e6  ErrMax=1e-4  UnitsV=kV  UnitsW=MW  buscounter=0  FunctionMessages=off  echomessages=off  EnableUseOfTLC=off  CurrentSourceSwitches=off  DisableSnubberDevices=off  DisableRonSwitches=off  DisableVfSwitches=off  DisplayEquations=off  AutomaticDiscreteSolvers=off  SolverType=Tustin/Backward Euler (TBE)  Interpol=off  ExternalGateDelay=off  methode=off  Ts=SampleTime  x0status=blocks  SPID=on  SwTol=0  HookPort=off  NonlinearTolerance=1e-4  nMaxIteration=100  ContinueOnMaxIteration=off  RestoreLinks=warning  ResistiveCurrentMeasurement=off  Frange=[0:2:500]  Ylog=off  Xlog=on  ShowGrid=off  save=off  variable=ZData  structure=0  ZoomFFT=off  StartTime=0.0  cycles=1  DisplayStyle=1  fundamental=60  FreqAxis=off  MaxFrequency=1000  frequencyindicesteady=1  RmsSteady=1  display=off
  wL : Gain  Gain=2*pi*50*1000e-6  SampleTime=SampleTime
  tag scope: PSSmodel=global, V_dc=global
  wires:
  Machine Signals/1(w) -> Machines/1  "w (pu)"
  Machine Signals/2(d_theta) -> Machines/2
  Machine Signals/3(Pa) -> Machines/3
  Machine Signals/4(Vt) -> Machines/4
  PSS model/1 -> [PSSmodel]
  Machine Signals/5(Stop) -> Stop simulation if loss of synchronism/1
  [Vd] -> Sum5/2
  [V_dc] -> Divide/2
  Alpha-Beta-Zero to dq1/1 -> Demux/1
  Bus Selector1/1 -> Product/1, [Vpv]  "<V_PV>"
  Gain5/1 -> Sum8/2
  "Power (3ph, Instantaneous)"/1 -> Gain1/1
  Gain2/1 -> [Qinv], Display2/1
  P&O/1(D) -> "PWM Generator (DC - DC) "/1
  [Irr] -> Gain7/1
  Repeating Sequence1/1 -> Mux2/2, PWM Generator (2-Level)/2
  [Vabc] -> "Power (3ph, Instantaneous)"/1
  Inverter Side V-I Measurement2/1 -> Scope2/1, [Vabc], Vpcc1_log/1
  Sum6/1 -> Gain6/1
  [Ipv] -> "PV ( V, I, P )"/3
  [Pinv] -> Mux5/2
  PID Controller2/1 -> [Id_ref], Scope5/1, Sum3/1
  Gain1/1 -> [Pinv], Display1/1
  [ILabc] -> Demux3/1
  [Irr] -> "PV ( V, I, P )4"/1
  Bus Selector1/2 -> Product/2, [Ipv]  "<I_PV>"
  IGBT/Diode1/1 -> E1/1
  Alpha-Beta-Zero to dq0/1 -> Demux1/1
  [Qinv] -> "PV ( V, I, P )2"/2
  Sum3/1 -> PID Controller3/1
  Mux3/1 -> "PV ( V, I, P )1"/1
  [Id] -> Mux6/2
  Gain/1 -> Mux4/1
  [Id_ref] -> Mux6/1
  Demux1/1 -> [Vd]
  Demux2/1 -> [Id]
  Irradiance (W/m2)/1 -> [Irr], PV Array1/1(S)
  Mux1/1 -> dq0 to abc/1
  PWM Generator (2-Level)/1 -> [PWM_inv]
  Constant1/1 -> PV Array1/2(TempC)
  [V_dc] -> Divide1/2
  Inverter Side V-I Measurement1/2 -> [Iabc], Scope1/2
  Mux5/1 -> "PV ( V, I, P )2"/1
  [V_dc] -> Mux3/1
  PID Controller5/1 -> Sum8/1
  [Vpv] -> "PV ( V, I, P )"/2
  Voltage Measurement1/1 -> [V_dc], "V_dc "/1
  Iq*/1 -> [Iq_ref], Sum7/1
  Sum4/1 -> Sum5/1
  Inverter Side V-I Measurement1/1 -> Scope1/1
  THD/1 -> Gain3/1
  "Power (3ph, Instantaneous)"/2 -> Gain2/1
  Gain3/1 -> [THDi]
  wL/1 -> Sum4/2
  Demux3/1 -> THD/1
  Divide/1 -> Mux1/1
  PID Controller3/1 -> Sum4/1
  [Vabc] -> abc to Alpha-Beta-Zero/1
  Gain4/1 -> Divide/1
  Gain7/1 -> Mux5/1
  Sum8/1 -> Sum6/1
  Inverter Side V-I Measurement2/2 -> Scope2/2, [ILabc], Ipcc1_log/1
  Sum1/1 -> PID Controller1/1
  [Vpv] -> P&O/1(Vpv)
  [Iq] -> Mux7/2
  [Vabc] -> abc to Alpha-Beta-Zero1/1
  [Iq] -> wL/1
  [Id] -> Sum3/2, Scope5/2
  "PWM Generator (DC - DC) "/1 -> [PWM_boost]
  Gain6/1 -> Divide1/1
  abc to Alpha-Beta-Zero1/1 -> Alpha-Beta-Zero to dq1/1
  [Id] -> Gain5/1
  abc to dq0/1 -> Demux2/1
  Vgq/1 -> Sum1/1
  Constant4/1 -> [V_dc_ref]
  PID Controller1/1 -> Integrator/1
  [Iq_ref] -> Mux7/1
  Product/1 -> Gain8/1, Scope/1
  [V_dc] -> Sum2/2
  abc to Alpha-Beta-Zero/1 -> Alpha-Beta-Zero to dq0/1
  Integrator/1 -> [wt], Alpha-Beta-Zero to dq1/2
  Mux6/1 -> "PV ( V, I, P )3"/1
  Sum5/1 -> Gain4/1
  dq0 to abc/1 -> Mux2/1, PWM Generator (2-Level)/1
  [Ppv] -> Mux4/2
  Divide1/1 -> Mux1/2
  Sum7/1 -> PID Controller5/1
  [Iq] -> Sum7/2
  [PWM_inv] -> Two-Level Converter/1
  [THDi] -> "PV ( V, I, P )2"/3
  [ILabc] -> "Power (3ph, Instantaneous)"/2
  [wt] -> abc to dq0/2, Alpha-Beta-Zero to dq0/2
  Demux2/2 -> [Iq]
  [Vq] -> Sum6/2
  Mux4/1 -> "PV ( V, I, P )"/1
  Mux7/1 -> "PV ( V, I, P )3"/2
  [PWM_boost] -> IGBT/Diode1/1
  [V_dc_ref] -> Sum2/1
  Mux2/1 -> Scope4/1
  PV Array1/1(m) -> Bus Selector1/1
  Demux1/2 -> [Vq]
  Sum2/1 -> PID Controller2/1
  [Ipv] -> P&O/2(Ipv)
  [V_dc_ref] -> Mux3/2
  [Irr] -> Gain/1
  Demux/2 -> Sum1/2
  [wt] -> dq0 to abc/2
  Gain8/1 -> [Ppv]
  [Iabc] -> abc to dq0/1
  [Vabc_5] -> Vabc5_log/1
  connections:
  Bus_2 18 KV/LConn2 -- Three-Phase Transformer (Two Windings)/RConn2
  18KV/230KV 6.25 %Z/LConn2 -- Bus_2 18 KV/RConn2
  18KV/230KV 6.25 %Z/RConn2 -- Bus_7 230 KV/LConn2
  Bus_2 18 KV/RConn1 -- Load Flow Bus7/LConn1 -- 18KV/230KV 6.25 %Z/LConn1
  Bus_2 18 KV/RConn3 -- 18KV/230KV 6.25 %Z/LConn3
  Bus_7 230 KV/LConn1 -- 18KV/230KV 6.25 %Z/RConn1
  18KV/230KV 6.25 %Z/RConn3 -- Bus_7 230 KV/LConn3
  Load Flow Bus8/LConn1 -- 13.8 KV/230 KV 5.86 %Z/LConn1 -- Bus_3 13.8 KV/LConn1
  13.8 KV/230 KV 5.86 %Z/LConn2 -- Bus_3 13.8 KV/LConn2
  13.8 KV/230 KV 5.86 %Z/LConn3 -- Bus_3 13.8 KV/LConn3
  Bus_1 16.5 KV/LConn1 -- Load Flow Bus/LConn1 -- "16.5 KV/230 KV 5.76 %Z     "/LConn1
  Bus_1 16.5 KV/LConn3 -- "16.5 KV/230 KV 5.76 %Z     "/LConn3
  Bus_1 16.5 KV/LConn2 -- "16.5 KV/230 KV 5.76 %Z     "/LConn2
  13.8 KV/230 KV 5.86 %Z/RConn1 -- Bus_9 230 KV/RConn1
  13.8 KV/230 KV 5.86 %Z/RConn2 -- Bus_9 230 KV/RConn2
  13.8 KV/230 KV 5.86 %Z/RConn3 -- Bus_9 230 KV/RConn3
  Bus_4 230 KV/LConn1 -- Load Flow Bus1/LConn1 -- "16.5 KV/230 KV 5.76 %Z     "/RConn1
  Bus_4 230 KV/LConn2 -- "16.5 KV/230 KV 5.76 %Z     "/RConn2
  Line 8 - 9/LConn1 -- load1/LConn1 -- Bus_8 230 KV/LConn1
  Bus_8 230 KV/LConn2 -- load1/LConn2 -- Line 8 - 9/LConn2
  Line 8 - 9/LConn3 -- load1/LConn3 -- Bus_8 230 KV/LConn3
  "16.5 KV/230 KV 5.76 %Z     "/RConn3 -- Bus_4 230 KV/LConn3
  "Line 4 - 5 "/LConn3 -- Three-Phase Breaker/LConn3 -- Bus_5 230 KV/RConn3 -- load2/LConn3
  " Line 4 - 6"/LConn1 -- load4/LConn1 -- Bus_6 230 KV/RConn1
  " Line 4 - 6"/LConn2 -- load4/LConn2 -- Bus_6 230 KV/RConn2
  " Line 4 - 6"/LConn3 -- load4/LConn3 -- Bus_6 230 KV/RConn3
  Line 7- 8/LConn1 -- Bus_7 230 KV/RConn1
  Line 7- 8/LConn2 -- Bus_7 230 KV/RConn2
  Bus_7 230 KV/RConn3 -- Line 7- 8/LConn3
  Bus_8 230 KV/RConn1 -- Load Flow Bus6/LConn1 -- Line 7- 8/RConn1
  Line 7- 8/RConn2 -- Bus_8 230 KV/RConn2
  Line 7- 8/RConn3 -- Bus_8 230 KV/RConn3
  Line 8 - 9/RConn2 -- Bus_9 230 KV/LConn2
  Line 8 - 9/RConn1 -- Bus_9 230 KV/LConn1
  Line 8 - 9/RConn3 -- Bus_9 230 KV/LConn3
  "Line 5 - 7 "/RConn1 -- Load Flow Bus2/LConn1 -- Bus_5 230 KV/LConn1
  "Line 5 - 7 "/RConn2 -- Bus_5 230 KV/LConn2
  "Line 5 - 7 "/RConn3 -- Bus_5 230 KV/LConn3
  "Line 5 - 7 "/LConn1 -- Load Flow Bus4/LConn1 -- Bus_7 230 KV/RConn6
  "Line 5 - 7 "/LConn2 -- Bus_7 230 KV/RConn5
  "Line 5 - 7 "/LConn3 -- Bus_7 230 KV/RConn4
  " Line 6 - 9"/RConn1 -- Load Flow Bus5/LConn1 -- Bus_9 230 KV/LConn4
  Bus_9 230 KV/LConn5 -- " Line 6 - 9"/RConn2
  Bus_6 230 KV/LConn1 -- Load Flow Bus3/LConn1 -- " Line 6 - 9"/LConn1
  Bus_6 230 KV/LConn2 -- " Line 6 - 9"/LConn2
  Bus_6 230 KV/LConn3 -- " Line 6 - 9"/LConn3
  " Line 6 - 9"/RConn3 -- Bus_9 230 KV/LConn6
  "Line 4 - 5 "/RConn2 -- Bus_4 230 KV/RConn2
  "Line 4 - 5 "/RConn1 -- Bus_4 230 KV/RConn1
  "Line 4 - 5 "/RConn3 -- Bus_4 230 KV/RConn3
  " Line 4 - 6"/RConn2 -- Bus_4 230 KV/RConn5
  " Line 4 - 6"/RConn1 -- Bus_4 230 KV/RConn4
  " Line 4 - 6"/RConn3 -- Bus_4 230 KV/RConn6
  G3/LConn1 -- Bus_3 13.8 KV/RConn1
  G3/LConn2 -- Bus_3 13.8 KV/RConn2
  G3/LConn3 -- Bus_3 13.8 KV/RConn3
  Three-Phase Transformer (Two Windings)/RConn3 -- Bus_2 18 KV/LConn3
  Bus_2 18 KV/LConn1 -- Three-Phase Transformer (Two Windings)/RConn1
  G1/LConn1 -- Bus_1 16.5 KV/RConn1
  G1/LConn2 -- Bus_1 16.5 KV/RConn2
  G1/LConn3 -- Bus_1 16.5 KV/RConn3
  L1/LConn1 -- C3/RConn1 -- PV Array1/RConn1
  Three-Phase Series RLC Branch1/RConn2 -- Three-Phase Series RLC Branch2/LConn2 -- Three-Phase Series RLC Branch3/LConn2
  Three-Phase Series RLC Branch1/RConn3 -- Three-Phase Series RLC Branch2/LConn3 -- Three-Phase Series RLC Branch3/LConn3
  Three-Phase Series RLC Branch1/RConn1 -- Three-Phase Series RLC Branch2/LConn1 -- Three-Phase Series RLC Branch3/LConn1
  C4/LConn1 -- PV Array1/RConn2 -- C3/LConn1 -- IGBT/Diode1/RConn1 -- Voltage Measurement1/LConn2 -- Two-Level Converter/RConn2
  C4/RConn1 -- Two-Level Converter/RConn1 -- Voltage Measurement1/LConn1 -- Diode1/RConn1
  L1/RConn1 -- Diode1/LConn1 -- IGBT/Diode1/LConn1
  Three-Phase Series RLC Branch3/RConn1 -- Three-Phase Series RLC Branch3/RConn2 -- Three-Phase Series RLC Branch3/RConn3 -- "Ground "/LConn1
  Inverter Side V-I Measurement1/LConn1 -- Two-Level Converter/LConn1
  Three-Phase Transformer (Two Windings)/LConn3 -- Inverter Side V-I Measurement2/RConn3
  Three-Phase Series RLC Branch1/LConn3 -- Inverter Side V-I Measurement1/RConn3
  Three-Phase Series RLC Branch1/LConn2 -- Inverter Side V-I Measurement1/RConn2
  Inverter Side V-I Measurement2/LConn2 -- Three-Phase Series RLC Branch2/RConn2
  Inverter Side V-I Measurement2/RConn1 -- Three-Phase Transformer (Two Windings)/LConn1
  Inverter Side V-I Measurement2/LConn3 -- Three-Phase Series RLC Branch2/RConn3
  Inverter Side V-I Measurement2/RConn2 -- Three-Phase Transformer (Two Windings)/LConn2
  Three-Phase Series RLC Branch1/LConn1 -- Inverter Side V-I Measurement1/RConn1
  Inverter Side V-I Measurement1/LConn3 -- Two-Level Converter/LConn3
  Inverter Side V-I Measurement1/LConn2 -- Two-Level Converter/LConn2
  Inverter Side V-I Measurement2/LConn1 -- Three-Phase Series RLC Branch2/RConn1
  Three-Phase Parallel RLC Load/LConn1 -- Three-Phase Breaker/RConn1
  Three-Phase Parallel RLC Load/LConn2 -- Three-Phase Breaker/RConn2
  Three-Phase Parallel RLC Load/LConn3 -- Three-Phase Breaker/RConn3
  load2/LConn1 -- "Line 4 - 5 "/LConn1 -- Three-Phase Breaker/LConn1 -- Bus_5 230 KV/RConn1
  load2/LConn2 -- "Line 4 - 5 "/LConn2 -- Three-Phase Breaker/LConn2 -- Bus_5 230 KV/RConn2
